simulink model "geo_pos_rate"  (Simulink 5.0)
settings: Solver=ode45  StartTime=0.0  StopTime=3600  RelTol=1e-3
undefined symbols (not defined in the file or in its folder): trate_east, trate_north
settings Model: Creator=mcarroll  LastModifiedBy=mcarroll  ExtModeAutoUpdateStatusClock=off

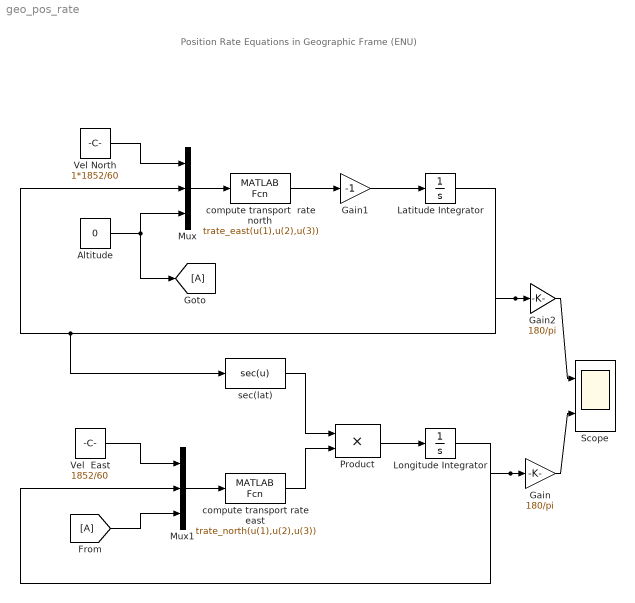
== system geo_pos_rate ==
  note: Position Rate Equations in Geographic Frame (ENU)
  Altitude : Constant  Value=0
  Gain : Gain  Gain=180/pi  SaturateOnIntegerOverflow=on
  Gain1 : Gain  Gain=-1  SaturateOnIntegerOverflow=on
  Gain2 : Gain  Gain=180/pi  SaturateOnIntegerOverflow=on
  Latitude Integrator : Integrator  InitialCondition=0*pi/180
  Longitude Integrator : Integrator
  Mux : Mux  Inputs=3
  Mux1 : Mux  Inputs=3
  Product : Product  SaturateOnIntegerOverflow=on
  Scope : Scope  NumInputPorts=2
      settings: YMin=-5~-5  YMax=5~5
  Vel  East : Constant  Value=1852/60
  Vel North : Constant  Value=1*1852/60
  compute transport rate east : MATLABFcn  MATLABFcn=trate_north(u(1),u(2),u(3))
  compute transport  rate north : MATLABFcn  MATLABFcn=trate_east(u(1),u(2),u(3))
  sec(lat) : MATLABFcn  MATLABFcn=sec(u)
  wires:
  Gain1/1 -> Latitude Integrator/1
  Mux/1 -> compute transport  rate north/1
  compute transport  rate north/1 -> Gain1/1
  Latitude Integrator/1 -> Mux/2, sec(lat)/1, Gain2/1
  Altitude/1 -> Mux/3, [A]
  Vel North/1 -> Mux/1
  sec(lat)/1 -> Product/1
  Mux1/1 -> compute transport rate east/1
  Product/1 -> Longitude Integrator/1
  Longitude Integrator/1 -> Mux1/2, Gain/1
  [A] -> Mux1/3
  Vel  East/1 -> Mux1/1
  compute transport rate east/1 -> Product/2
  Gain/1 -> Scope/2
  Gain2/1 -> Scope/1
